simulink model "ME486C_Dyno_DAQ_Quality_Development"  (R2025a)
settings: Solver=FixedStepAuto  StartTime=0.0  StopTime=inf  FixedStep=0.02  RelTol=1e-3  EnableMultiTasking=on
libraries: arduinolib x24, simulink x19
(part 2 of 2)

== system ME486C_Dyno_DAQ_Quality_Development/Sensor Acquisition/Load Cell-NAU7802/NAU7802 Initialization/Flush ADC Readings ==
  Enable : EnablePort
  Add : Sum
  Constant : Constant  OutDataTypeStr=uint8
  I2C Read : arduinolib/I2C Read  I2CModule=0  Mode=Master  SlaveAddress=hex2dec('2A')  SlaveByteOrder=BigEndian  Direction=Receiver  RegisterAddressMode=on  RegisterAddress=hex2dec('12')  SlaveDataType=uint8  DataLength=3  NoAck=off  RepeatedStart=off  OutputStatus=on  blockPlatform=ARDUINO  SampleTime=0.02
  Unit Delay : UnitDelay  SampleTime=-1  HasFrameUpgradeWarning=on
  flush_count : Outport
  wires:
  Add/1 -> flush_count/1, Unit Delay/1
  Unit Delay/1 -> Add/1
  Constant/1 -> Add/2

== system ME486C_Dyno_DAQ_Quality_Development/Sensor Acquisition/Load Cell-NAU7802/NAU7802 Initialization/Power up ==
  Enable : EnablePort
  Constant : Constant  Value=6  OutDataTypeStr=uint8
  I2C Write : arduinolib/I2C Write  I2CModule=0  Mode=Master  SlaveAddress=hex2dec('2A')  SlaveByteOrder=BigEndian  Direction=Transmitter  RegisterAddressMode=on  RegisterAddress=hex2dec('00')  SlaveDataType=uint8  DataLength=1  NoAck=off  RepeatedStart=off  OutputStatus=on  blockPlatform=ARDUINO
  wires:
  Constant/1 -> I2C Write/1

== system ME486C_Dyno_DAQ_Quality_Development/Sensor Acquisition/Load Cell-NAU7802/NAU7802 Initialization/Reset Assert ==
  Enable : EnablePort
  Constant : Constant  OutDataTypeStr=uint8
  I2C Write : arduinolib/I2C Write  I2CModule=0  Mode=Master  SlaveAddress=hex2dec('2A')  SlaveByteOrder=BigEndian  Direction=Transmitter  RegisterAddressMode=on  RegisterAddress=hex2dec('00')  SlaveDataType=uint8  DataLength=1  NoAck=off  RepeatedStart=off  OutputStatus=on  blockPlatform=ARDUINO
  wires:
  Constant/1 -> I2C Write/1

== system ME486C_Dyno_DAQ_Quality_Development/Sensor Acquisition/Load Cell-NAU7802/NAU7802 Initialization/Reset Release ==
  Enable : EnablePort
  Constant : Constant  Value=0  OutDataTypeStr=uint8
  I2C Write : arduinolib/I2C Write  I2CModule=0  Mode=Master  SlaveAddress=hex2dec('2A')  SlaveByteOrder=BigEndian  Direction=Transmitter  RegisterAddressMode=on  RegisterAddress=hex2dec('00')  SlaveDataType=uint8  DataLength=1  NoAck=off  RepeatedStart=off  OutputStatus=off  blockPlatform=ARDUINO
  wires:
  Constant/1 -> I2C Write/1

== matlab function ME486C_Dyno_DAQ_Quality_Development/Signal Quality Mentor/MATLAB Function ==
  data: Force_N input; Force_Quality_OK output; RPM input; RPM_Quality_OK output; Temp_In_C input; Temp_Out_C input; RPM_Valid input; RPM_Timeout input; Temp_In_Valid input; Temp_In_Fault input; Temp_Out_Valid input; Temp_Out_Fault input; Flow_Lmin input; Flow_Valid input; Temp_In_Quality_OK output; Temp_Out_Quality_OK output; Flow_Quality_OK output; All_Sensors_OK output; Quality_Fault_Code output; Quality_Warning output

function [Force_Quality_OK, RPM_Quality_OK, ...
    Temp_In_Quality_OK, Temp_Out_Quality_OK, ...
    Flow_Quality_OK, All_Sensors_OK, ...
    Quality_Fault_Code, Quality_Warning] = ...
    Quality_Check_Core(Force_N, RPM, Temp_In_C, Temp_Out_C, ...
    RPM_Valid, RPM_Timeout, Temp_In_Valid, Temp_In_Fault, ...
    Temp_Out_Valid, Temp_Out_Fault, Flow_Lmin, Flow_Valid)
%#codegen
% =========================================================
% DynoForge - Signal Quality Monitor V2
% Model: ME486C_Dyno_DAQ_Quality_Development
%
% Inputs:  12
% Outputs: 8
%
% Functions:
% 1. Numerical signal validation
% 2. Sensor validity and fault flag checking
% 3. Individual sensor quality monitoring
% 4. Combined sensor quality evaluation
% 5. Quality fault bitmask generation
%
% IMPORTANT:
% Preliminary thresholds only.
% Diagnostic monitoring, not a physical safety interlock.
% =========================================================

%% 1. Convert measurement inputs to double

force = double(Force_N);
rpm_value = double(RPM);

temp_in = double(Temp_In_C);
temp_out = double(Temp_Out_C);

flow_value = double(Flow_Lmin);

%% 2. Normalize validity and fault flags

rpm_valid_flag = (double(RPM_Valid) ~= 0);
rpm_timeout_flag = (double(RPM_Timeout) ~= 0);

temp_in_valid_flag = (double(Temp_In_Valid) ~= 0);
temp_in_fault_flag = (double(Temp_In_Fault) ~= 0);

temp_out_valid_flag = (double(Temp_Out_Valid) ~= 0);
temp_out_fault_flag = (double(Temp_Out_Fault) ~= 0);

flow_valid_flag = (double(Flow_Valid) ~= 0);

%% 3. Force quality check

force_finite = isfinite(force);

force_range_ok = ...
    (force >= -2000.0) && ...
    (force <= 2000.0);

Force_Quality_OK = logical( ...
    force_finite && ...
    force_range_ok);

%% 4. RPM quality check

rpm_finite = isfinite(rpm_value);

rpm_range_ok = ...
    (rpm_value >= 0.0) && ...
    (rpm_value <= 11000.0);

RPM_Quality_OK = logical( ...
    rpm_finite && ...
    rpm_range_ok && ...
    rpm_valid_flag && ...
    ~rpm_timeout_flag);

%% 5. Inlet temperature quality check

temp_in_finite = isfinite(temp_in);

temp_in_range_ok = ...
    (temp_in >= -20.0) && ...
    (temp_in <= 150.0);

Temp_In_Quality_OK = logical( ...
    temp_in_finite && ...
    temp_in_range_ok && ...
    temp_in_valid_flag && ...
    ~temp_in_fault_flag);

%% 6. Outlet temperature quality check

temp_out_finite = isfinite(temp_out);

temp_out_range_ok = ...
    (temp_out >= -20.0) && ...
    (temp_out <= 150.0);

Temp_Out_Quality_OK = logical( ...
    temp_out_finite && ...
    temp_out_range_ok && ...
    temp_out_valid_flag && ...
    ~temp_out_fault_flag);

%% 7. Flow quality check

flow_finite = isfinite(flow_value);

flow_range_ok = ...
    (flow_value >= 0.0) && ...
    (flow_value <= 100.0);

Flow_Quality_OK = logical( ...
    flow_finite && ...
    flow_range_ok && ...
    flow_valid_flag);

%% 8. Overall sensor quality

All_Sensors_OK = logical( ...
    Force_Quality_OK && ...
    RPM_Quality_OK && ...
    Temp_In_Quality_OK && ...
    Temp_Out_Quality_OK && ...
    Flow_Quality_OK);

%% 9. Fault code generation

% Fault bitmask:
% 1  = Force invalid
% 2  = RPM invalid
% 4  = Inlet temperature invalid
% 8  = Outlet temperature invalid
% 16 = Flow invalid
%
% Multiple faults are combined using bitwise OR.
% Maximum code = 31.

Quality_Fault_Code = uint16(0);

if ~Force_Quality_OK
    Quality_Fault_Code = bitor( ...
        Quality_Fault_Code, uint16(1));
end

if ~RPM_Quality_OK
    Quality_Fault_Code = bitor( ...
        Quality_Fault_Code, uint16(2));
end

if ~Temp_In_Quality_OK
    Quality_Fault_Code = bitor( ...
        Quality_Fault_Code, uint16(4));
end

if ~Temp_Out_Quality_OK
    Quality_Fault_Code = bitor( ...
        Quality_Fault_Code, uint16(8));
end

if ~Flow_Quality_OK
    Quality_Fault_Code = bitor( ...
        Quality_Fault_Code, uint16(16));
end

%% 10. Quality warning

Quality_Warning = logical(~All_Sensors_OK);

end

== matlab function ME486C_Dyno_DAQ_Quality_Development/Calibration Manager/Calibration_Status_Core ==
  data: LoadCell_Scale input; LoadCell_Param_OK output; LoadCell_Zero input; RPM_Pulses_Per_Rev input; Temp_In_Offset input; Temp_Out_Offset input; Flow_K_Factor input; RPM_Param_OK output; Temp_In_Param_OK output; Temp_Out_Param_OK output; Flow_Param_OK output; All_Params_Valid output; Calibration_Complete output; Calibration_Fault_Code output; Calibration_Confirmed input

function [LoadCell_Param_OK, RPM_Param_OK, ...
    Temp_In_Param_OK, Temp_Out_Param_OK, ...
    Flow_Param_OK, All_Params_Valid, ...
    Calibration_Complete, Calibration_Fault_Code] = ...
    Calibration_Status_Core(LoadCell_Scale, LoadCell_Zero, ...
    RPM_Pulses_Per_Rev, Temp_In_Offset, ...
    Temp_Out_Offset, Flow_K_Factor, Calibration_Confirmed)
%#codegen
% ============================================================
% DynoForge - Calibration Manager
% Calibration Status Core
% NAU ME486C Engine Dynamometer
%
% PURPOSE:
% 1. Validate sensor calibration parameters.
% 2. Generate calibration status signals.
% 3. Generate a calibration fault bitmask.
% 4. Distinguish valid parameters from confirmed calibration.
%
% NOTE:
% Flow K-factor = 50 pulses/L is a temporary test value.
% Calibration_Confirmed must remain false until actual
% calibration has been completed and verified.
%
% Fault code:
%   1  = Load cell parameter invalid
%   2  = RPM parameter invalid
%   4  = Inlet temperature parameter invalid
%   8  = Outlet temperature parameter invalid
%   16 = Flow K-factor invalid
% ============================================================

%% 1. Convert inputs to double

lc_scale = double(LoadCell_Scale);
lc_zero = double(LoadCell_Zero);

rpm_ppr = double(RPM_Pulses_Per_Rev);

tin_offset = double(Temp_In_Offset);
tout_offset = double(Temp_Out_Offset);

flow_k = double(Flow_K_Factor);

%% 2. Load cell parameter validation

LoadCell_Param_OK = logical( ...
    isfinite(lc_scale) && ...
    lc_scale > 0.0 && ...
    isfinite(lc_zero));

%% 3. RPM parameter validation

RPM_Param_OK = logical( ...
    isfinite(rpm_ppr) && ...
    rpm_ppr >= 1.0 && ...
    rpm_ppr == floor(rpm_ppr));

%% 4. Inlet temperature parameter validation

Temp_In_Param_OK = logical( ...
    isfinite(tin_offset) && ...
    abs(tin_offset) <= 20.0);

%% 5. Outlet temperature parameter validation

Temp_Out_Param_OK = logical( ...
    isfinite(tout_offset) && ...
    abs(tout_offset) <= 20.0);

%% 6. Flow K-factor validation

Flow_Param_OK = logical( ...
    isfinite(flow_k) && ...
    flow_k > 0.0);

%% 7. Combined parameter validity

All_Params_Valid = logical( ...
    LoadCell_Param_OK && ...
    RPM_Param_OK && ...
    Temp_In_Param_OK && ...
    Temp_Out_Param_OK && ...
    Flow_Param_OK);

%% 8. Calibration confirmation

Calibration_Complete = logical( ...
    All_Params_Valid && ...
    logical(Calibration_Confirmed));

%% 9. Calibration fault bitmask

Calibration_Fault_Code = uint16(0);

if ~LoadCell_Param_OK
    Calibration_Fault_Code = bitor( ...
        Calibration_Fault_Code, uint16(1));
end

if ~RPM_Param_OK
    Calibration_Fault_Code = bitor( ...
        Calibration_Fault_Code, uint16(2));
end

if ~Temp_In_Param_OK
    Calibration_Fault_Code = bitor( ...
        Calibration_Fault_Code, uint16(4));
end

if ~Temp_Out_Param_OK
    Calibration_Fault_Code = bitor( ...
        Calibration_Fault_Code, uint16(8));
end

if ~Flow_Param_OK
    Calibration_Fault_Code = bitor( ...
        Calibration_Fault_Code, uint16(16));
end

end

== matlab function ME486C_Dyno_DAQ_Quality_Development/Alarm Manager/Alarm_Logic_Core ==
  data: SQ_Quality_Warning input; Alarm_Active output; SQ_Quality_Fault_Code input; CAL_All_Params_Valid input; CAL_Calibration_Complete input; Shutdown_Request input; Alarm_Level output; Alarm_Code output; Sensor_Alarm output; Calibration_Alarm output; Shutdown_Alarm output

function [Alarm_Active, Alarm_Level, Alarm_Code, ...
    Sensor_Alarm, Calibration_Alarm, ...
    Shutdown_Alarm] = Alarm_Logic_Core( ...
    SQ_Quality_Warning, SQ_Quality_Fault_Code, ...
    CAL_All_Params_Valid, CAL_Calibration_Complete, ...
    Shutdown_Request)
%#codegen
% DynoForge - Alarm Manager
%
% Alarm levels:
% 0 = Normal
% 1 = Advisory (calibration incomplete)
% 2 = Warning (sensor quality or invalid parameters)
% 3 = Critical (existing shutdown request)
%
% Alarm code bitmask:
% 1 = Sensor quality warning
% 2 = Calibration parameters invalid
% 4 = Calibration incomplete
% 8 = Shutdown requested
%
% This block only reports alarms.
% It does NOT control the safety shutdown system.

%% Input conversion
sq_warning = logical(SQ_Quality_Warning);
sq_code = uint16(SQ_Quality_Fault_Code);

cal_valid = logical(CAL_All_Params_Valid);
cal_complete = logical(CAL_Calibration_Complete);

shutdown = logical(Shutdown_Request);

%% Alarm categories
Sensor_Alarm = sq_warning || (sq_code ~= uint16(0));

Calibration_Alarm = ~cal_valid || ~cal_complete;

Shutdown_Alarm = shutdown;

%% Alarm code
Alarm_Code = uint16(0);

if Sensor_Alarm
    Alarm_Code = bitor(Alarm_Code, uint16(1));
end

if ~cal_valid
    Alarm_Code = bitor(Alarm_Code, uint16(2));
end

if ~cal_complete
    Alarm_Code = bitor(Alarm_Code, uint16(4));
end

if Shutdown_Alarm
    Alarm_Code = bitor(Alarm_Code, uint16(8));
end

%% Highest active alarm level
Alarm_Level = uint8(0);

if ~cal_complete
    Alarm_Level = uint8(1);
end

if Sensor_Alarm || ~cal_valid
    Alarm_Level = uint8(2);
end

if Shutdown_Alarm
    Alarm_Level = uint8(3);
end

Alarm_Active = Alarm_Code ~= uint16(0);

end

== matlab function ME486C_Dyno_DAQ_Quality_Development/Test Sequence Controller/Test_Sequence_Core ==
  data: Start_Command input; Test_State output; Stop_Command input; Reset_Command input; Run_Permit input; Shutdown_Request input; SQ_All_Sensors_OK input; CAL_All_Params_Valid input; CAL_Calibration_Complete input; Alarm_Level input; Test_Active output; Test_Ready output; Test_Fault_Latched output; Start_Accepted output; Stop_Active output; Sequence_Permit output; State_Changed output

function [Test_State, Test_Active, Test_Ready, ...
    Test_Fault_Latched, Start_Accepted, ...
    Stop_Active, Sequence_Permit, State_Changed] = ...
    Test_Sequence_Core( ...
    Start_Command, Stop_Command, Reset_Command, ...
    Run_Permit, Shutdown_Request, ...
    SQ_All_Sensors_OK, CAL_All_Params_Valid, ...
    CAL_Calibration_Complete, Alarm_Level)
%#codegen
% ============================================================
% DynoForge - Test Sequence Controller
% NAU ME486C Engine Dynamometer
%
% STATE DEFINITIONS
% 0 = IDLE
% 1 = READY
% 2 = RUNNING
% 3 = STOPPING
% 4 = FAULT
%
% SOFTWARE SUPERVISORY LOGIC ONLY
% Does not actuate engine, brake, or physical E-stop.
% ============================================================

persistent state

if isempty(state)
    state = uint8(0);
end

%% 1. Convert inputs

startCmd = logical(Start_Command);
stopCmd = logical(Stop_Command);
resetCmd = logical(Reset_Command);

runPermit = logical(Run_Permit);
shutdown = logical(Shutdown_Request);

sensorsOK = logical(SQ_All_Sensors_OK);
paramsValid = logical(CAL_All_Params_Valid);
calComplete = logical(CAL_Calibration_Complete);

alarm = uint8(Alarm_Level);

%% 2. Define conditions

readyConditions = ...
    runPermit && ...
    ~shutdown && ...
    sensorsOK && ...
    paramsValid && ...
    calComplete && ...
    (alarm < uint8(2));

criticalFault = ...
    shutdown || ...
    (alarm >= uint8(3));

operatingFault = ...
    ~runPermit || ...
    ~sensorsOK || ...
    ~paramsValid || ...
    ~calComplete || ...
    (alarm >= uint8(2));

%% 3. Save previous state

previousState = state;

%% 4. State machine

switch state

    case uint8(0)
        % IDLE
        if criticalFault
            state = uint8(4);

        elseif startCmd && ~stopCmd && ...
                ~resetCmd && readyConditions
            state = uint8(1);
        end

    case uint8(1)
        % READY
        if criticalFault || operatingFault
            state = uint8(4);

        elseif stopCmd || ~startCmd
            state = uint8(0);

        else
            state = uint8(2);
        end

    case uint8(2)
        % RUNNING
        if criticalFault || operatingFault
            state = uint8(4);

        elseif stopCmd || ~startCmd
            state = uint8(3);
        end

    case uint8(3)
        % STOPPING
        if criticalFault
            state = uint8(4);

        elseif ~stopCmd && ~startCmd
            state = uint8(0);
        end

    case uint8(4)
        % FAULT - latched
        if resetCmd && ...
                ~startCmd && ...
                ~stopCmd && ...
                ~criticalFault && ...
                ~operatingFault
            state = uint8(0);
        end

    otherwise
        state = uint8(4);

end

%% 5. Outputs

Test_State = state;

Test_Active = (state == uint8(2));

Test_Ready = (state == uint8(1));

Test_Fault_Latched = (state == uint8(4));

Start_Accepted = ...
    (previousState == uint8(0)) && ...
    (state == uint8(1));

Stop_Active = (state == uint8(3));

Sequence_Permit = ...
    (state == uint8(2)) && ...
    readyConditions && ...
    ~criticalFault;

State_Changed = (state ~= previousState);

end

== matlab function ME486C_Dyno_DAQ_Quality_Development/Sensor Acquisition/Temperature In-Max31865/MAX31865_Temperature Conversion ==
  data: rtdBytes input; Temp_In_C output; faultBytes input; Temp_In_Valid output; Temp_In_Fault output; Temp_In_Raw output

function [Temp_In_C, Temp_In_Valid, Temp_In_Fault, Temp_In_Raw] = fcn(rtdBytes, faultBytes)
%#codegen
% MAX31865 Pt100 RTD - Inlet Water Temperature
% 3-wire RTD
% Rref = 430 ohms
% IEC 60751 Callendar-Van Dusen, positive temperature branch
%
% Expected SPI RX:
% rtdBytes   = uint8 vector [dummy, RTD_MSB, RTD_LSB]
% faultBytes = uint8 vector [dummy, fault_status]

RREF = 430.0;
R0   = 100.0;

A = 3.9083e-3;
B = -5.775e-7;

Temp_In_C = 0.0;
Temp_In_Valid = false;
Temp_In_Fault = uint8(0);
Temp_In_Raw = uint16(0);

% Extract SPI data bytes
msb = uint16(rtdBytes(2));
lsb = uint16(rtdBytes(3));

% Combine RTD register bytes
raw16 = bitor(bitshift(msb, 8), lsb);

% Bit 0 is MAX31865 fault flag
faultBit = bitand(raw16, uint16(1));

% 15-bit RTD ADC value
rtdCode = bitshift(raw16, -1);
Temp_In_Raw = rtdCode;

% Read fault status register
Temp_In_Fault = uint8(faultBytes(2));

% Convert RTD ADC code to resistance
Rtd = double(rtdCode) * RREF / 32768.0;

% Positive-temperature Callendar-Van Dusen inversion
ratio = Rtd / R0;

discriminant = A*A - 4.0*B*(1.0-ratio);

if discriminant >= 0.0

    temperature = (-A + sqrt(discriminant)) / (2.0*B);

    if isfinite(temperature) && ...
       temperature >= 0.0 && ...
       temperature <= 200.0 && ...
       Temp_In_Fault == uint8(0) && ...
       faultBit == uint16(0)

        Temp_In_C = temperature;
        Temp_In_Valid = true;

    end
end
end

== matlab function ME486C_Dyno_DAQ_Quality_Development/Sensor Acquisition/RPM-Hall sensor/Pulse counter/RPM_Period measurement ==
  data: RPM_Event output; RPM_Valid output

function [RPM_Event, RPM_Valid] = fcn()
%#codegen

% Arduino UNO R4 Minima
% Hall sensor: 10 pulses per revolution
% Hardware timing using micros()

persistent tbuf idx filled

if isempty(tbuf)
    tbuf = zeros(1,10,'uint32');
    idx = uint8(1);
    filled = uint8(0);
end

% Read microsecond timestamp
tNow = uint32(0);

if coder.target('Rtw')
    coder.cinclude('Arduino.h');
    tNow = coder.ceval('micros');
else
    % Desktop simulation placeholder only
    % NOT a real Hall pulse timestamp
    tNow = uint32(0);
end

% Read timestamp from 10 calls ago
tOld = tbuf(double(idx));

% Store current timestamp
tbuf(double(idx)) = tNow;

% Update circular buffer
if idx >= 10
    idx = uint8(1);
else
    idx = idx + uint8(1);
end

% Wait until 10 timestamps are collected
if filled < 10
    filled = filled + uint8(1);
    RPM_Event = 0.0;
    RPM_Valid = false;
    return;
end

% Handle uint32 timer rollover
if tNow >= tOld
    dt_us = tNow - tOld;
else
    dt_us = uint32(4294967295) - tOld + ...
            tNow + uint32(1);
end

% Calculate RPM
if dt_us > 0
    RPM_Event = 60000000.0 / double(dt_us);
    RPM_Valid = true;
else
    RPM_Event = 0.0;
    RPM_Valid = false;
end

end

== matlab function ME486C_Dyno_DAQ_Quality_Development/Sensor Acquisition/Temperature Out-Max31865/MAX31865_Temperature Conversion ==
  data: rtdBytes input; Temp_Out_C output; faultBytes input; Temp_Out_Valid output; Temp_Out_Fault output; Temp_Out_Raw output

function [Temp_Out_C, Temp_Out_Valid, Temp_Out_Fault, Temp_Out_Raw] = fcn(rtdBytes, faultBytes)
%#codegen
% DynoForge MAX31865 - Outlet Water Temperature
% Sensor: 3-wire Pt100 RTD
% Reference resistor: 430 ohms
% IEC 60751 Callendar-Van Dusen equation
%
% Expected SPI RX:
% rtdBytes   = uint8([dummy, RTD_MSB, RTD_LSB])
% faultBytes = uint8([dummy, fault_status])

% RTD parameters
RREF = 430.0;
R0   = 100.0;

A = 3.9083e-3;
B = -5.775e-7;

% Initialize outputs
Temp_Out_C = 0.0;
Temp_Out_Valid = false;
Temp_Out_Fault = uint8(0);
Temp_Out_Raw = uint16(0);

% Extract RTD bytes
msb = uint16(rtdBytes(2));
lsb = uint16(rtdBytes(3));

% Combine 16-bit register data
raw16 = bitor(bitshift(msb, 8), lsb);

% MAX31865 fault flag
faultBit = bitand(raw16, uint16(1));

% Extract 15-bit RTD ADC code
rtdCode = bitshift(raw16, -1);
Temp_Out_Raw = rtdCode;

% Read fault status register
Temp_Out_Fault = uint8(faultBytes(2));

% Convert ADC code to RTD resistance
Rtd = double(rtdCode) * RREF / 32768.0;

% Positive-temperature CVD inversion
ratio = Rtd / R0;
discriminant = A*A - 4.0*B*(1.0-ratio);

if discriminant >= 0.0

    temperature = (-A + sqrt(discriminant)) / (2.0*B);

    if isfinite(temperature) && ...
       temperature >= 0.0 && ...
       temperature <= 200.0 && ...
       Temp_Out_Fault == uint8(0) && ...
       faultBit == uint16(0)

        Temp_Out_C = temperature;
        Temp_Out_Valid = true;

    end
end

end

== matlab function ME486C_Dyno_DAQ_Quality_Development/Sensor Acquisition/Water_flow UFM02/Flow Calibration ==
  data: Flow_Hz input; Flow_Lmin output; K_Pulses_Per_Liter input; Flow_Valid output
function [Flow_Lmin, Flow_Valid] = fcn(Flow_Hz, K_Pulses_Per_Liter)
%#codegen
% DynoForge UFM-02 Flow Conversion
% Flow_Hz unit: pulses per second (Hz)
% K unit: pulses per liter
% Flow_Lmin unit: liters per minute (L/min)
% Flow_Valid: double flag (1.0 = valid, 0.0 = invalid)

% Convert inputs to double to avoid fixed-point division errors
flow_hz = double(Flow_Hz);
k_factor = double(K_Pulses_Per_Liter);

% Initialize outputs explicitly as double
Flow_Lmin = double(NaN);
Flow_Valid = 0.0;

% Validate pulse frequency
if ~isfinite(flow_hz) || flow_hz < 0.0
    return;
end

% Validate calibration factor
if ~isfinite(k_factor) || k_factor <= 0.0
    return;
end

% Convert pulse frequency to volumetric flow rate
Flow_Lmin = 60.0 * flow_hz / k_factor;

% Numerical inputs are valid
Flow_Valid = 1.0;

end

== matlab function ME486C_Dyno_DAQ_Quality_Development/fault detection/MATLAB Function ==
  data: OverTemp_Condition input; OverTemp_Trip output; Temp_Sensor_Fault input; Cooling_Data_Fault input; Low_Flow_Condition input; Overspeed_Condition input; RPM_Timeout input; RPM_VALID input; EStop_Fault input; Safety_Chain_Fault input; Config_Not_Ready input; Engine_Run_Command input; Reset_Command input; Temp_Sensor_Trip output; Cooling_Data_Trip output; Low_Flow_Trip output; Overspeed_Trip output; RPM_Loss_Trip output; Start_Timeout_Fault output; EStop_Trip output; Safety_Chain_Trip output; Any_Trip output; Trip_Latched output; Shutdown_Request output; Run_Permit output; Controller_State output; Reset_Accepted output; Fault_Code output

function [OverTemp_Trip, Temp_Sensor_Trip, Cooling_Data_Trip, ...
          Low_Flow_Trip, Overspeed_Trip, RPM_Loss_Trip, ...
          Start_Timeout_Fault, EStop_Trip, Safety_Chain_Trip, ...
          Any_Trip, Trip_Latched, Shutdown_Request, Run_Permit, ...
          Controller_State, Reset_Accepted, Fault_Code] = ...
          fcn(OverTemp_Condition, Temp_Sensor_Fault, ...
              Cooling_Data_Fault, Low_Flow_Condition, ...
              Overspeed_Condition, RPM_Timeout, RPM_VALID, ...
              EStop_Fault, Safety_Chain_Fault, Config_Not_Ready, ...
              Engine_Run_Command, Reset_Command)

%#codegen
%
% DynoForge Fault Detection and Automatic Shutdown
% Software prototype - NOT validated for engine operation.
%
% Controller states:
% 0 = STOPPED
% 1 = PRESTART
% 2 = STARTING
% 3 = RUNNING
% 4 = TRIPPED
%
% Sample time: 0.02 seconds
%
% IMPORTANT:
% - All safety thresholds must be validated.
% - Independent hardware emergency stop is required.
% - Shutdown_Request is a software request only.

persistent state latch start_count prev_reset prev_run

if isempty(state)
    state = uint8(0);
    latch = true;
    start_count = uint32(0);
    prev_reset = false;
    prev_run = false;
end

%% 1. Input conversion

run_cmd = (Engine_Run_Command ~= 0);
reset_cmd = (Reset_Command ~= 0);

rpm_valid = (RPM_VALID ~= 0);
rpm_timeout = (RPM_Timeout ~= 0);

estop_fault = (EStop_Fault ~= 0);
safety_fault = (Safety_Chain_Fault ~= 0);
config_fault = (Config_Not_Ready ~= 0);

temp_fault = (Temp_Sensor_Fault ~= 0);
cooling_fault = (Cooling_Data_Fault ~= 0);

overtemp = (OverTemp_Condition ~= 0);
low_flow = (Low_Flow_Condition ~= 0);
overspeed = (Overspeed_Condition ~= 0);

%% 2. Edge detection

reset_edge = reset_cmd && ~prev_reset;
run_edge = run_cmd && ~prev_run;

prev_reset = reset_cmd;
prev_run = run_cmd;

%% 3. Default fault outputs

OverTemp_Trip = overtemp;
Temp_Sensor_Trip = temp_fault;
Cooling_Data_Trip = cooling_fault;

Low_Flow_Trip = low_flow;
Overspeed_Trip = overspeed;

RPM_Loss_Trip = false;
Start_Timeout_Fault = false;

EStop_Trip = estop_fault;
Safety_Chain_Trip = safety_fault;

Reset_Accepted = false;

%% 4. Software diagnostic timing
%
% TEST VALUE ONLY:
% 250 samples * 0.02 s = 5 seconds.
%
% Must be approved for the actual engine.

START_TIMEOUT_SAMPLES = uint32(250);

%% 5. Active critical fault checks

critical_fault = ...
    OverTemp_Trip || ...
    Temp_Sensor_Trip || ...
    Cooling_Data_Trip || ...
    Low_Flow_Trip || ...
    Overspeed_Trip || ...
    EStop_Trip || ...
    Safety_Chain_Trip;

%% 6. Controller state machine

switch state

    case uint8(0)
        % STOPPED
        % Startup is inhibited until a valid manual reset.
        start_count = uint32(0);

        if critical_fault
            latch = true;
            state = uint8(4);

        elseif reset_edge && ~run_cmd && ~config_fault
            latch = false;
            Reset_Accepted = true;

        elseif run_edge && ~latch && ~config_fault
            state = uint8(1);
        end

    case uint8(1)
        % PRESTART
        % Check required conditions before starting.

        if critical_fault || config_fault
            latch = true;
            state = uint8(4);

        elseif ~run_cmd
            state = uint8(0);

        else
            start_count = uint32(0);
            state = uint8(2);
        end

    case uint8(2)
        % STARTING

        if critical_fault || config_fault
            latch = true;
            state = uint8(4);

        elseif ~run_cmd
            state = uint8(0);

        elseif rpm_valid && ~rpm_timeout
            start_count = uint32(0);
            state = uint8(3);

        else
            if start_count < START_TIMEOUT_SAMPLES
                start_count = start_count + uint32(1);
            end

            if start_count >= START_TIMEOUT_SAMPLES
                Start_Timeout_Fault = true;
                latch = true;
                state = uint8(4);
            end
        end

    case uint8(3)
        % RUNNING

        RPM_Loss_Trip = rpm_timeout || ~rpm_valid;

        if critical_fault || RPM_Loss_Trip || config_fault
            latch = true;
            state = uint8(4);

        elseif ~run_cmd
            state = uint8(0);
        end

    case uint8(4)
        % TRIPPED
        % Fault remains latched until manual reset.

        latch = true;

        if reset_edge && ...
           ~run_cmd && ...
           ~critical_fault && ...
           ~config_fault

            latch = false;
            Reset_Accepted = true;
            state = uint8(0);
        end

    otherwise
        % Invalid state -> trip
        latch = true;
        state = uint8(4);

end

%% 7. Any_Trip
%
% Config_Not_Ready inhibits operation.
% It is included in the overall unsafe condition.

Any_Trip = ...
    critical_fault || ...
    RPM_Loss_Trip || ...
    Start_Timeout_Fault || ...
    config_fault;

%% 8. Shutdown and run permission

Trip_Latched = latch;

Shutdown_Request = ...
    latch || Any_Trip || (state == uint8(4));

Run_Permit = ...
    ~Shutdown_Request && ...
    ~config_fault && ...
    ~estop_fault && ...
    ~safety_fault && ...
    (state == uint8(1) || ...
     state == uint8(2) || ...
     state == uint8(3));

%% 9. Controller state output

Controller_State = state;

%% 10. Fault code
%
% Priority-based diagnostic code.
% Individual fault outputs remain available.

Fault_Code = uint8(0);

if EStop_Trip
    Fault_Code = uint8(1);

elseif Safety_Chain_Trip
    Fault_Code = uint8(2);

elseif Overspeed_Trip
    Fault_Code = uint8(3);

elseif OverTemp_Trip
    Fault_Code = uint8(4);

elseif Low_Flow_Trip
    Fault_Code = uint8(5);

elseif Temp_Sensor_Trip
    Fault_Code = uint8(6);

elseif Cooling_Data_Trip
    Fault_Code = uint8(7);

elseif RPM_Loss_Trip
    Fault_Code = uint8(8);

elseif Start_Timeout_Fault
    Fault_Code = uint8(9);

elseif config_fault
    Fault_Code = uint8(10);

end

end
